simulink model "gnc_PathTracker"  (R2026b)
settings: Solver=VariableStepAuto
values from neighbouring files (symbols this model uses):
  Ts = prm.Ts    [gnc_missionFSM.m]    (also in gnc_mpcPlantUpdate.m)
undefined symbols (not defined in the file or in its folder): P
libraries: robotalgslib x1, mpclib x1, drivingvehiclecontroller x1, simulink x1
settings Model: Creator=aomar  LastModifiedBy=aomar

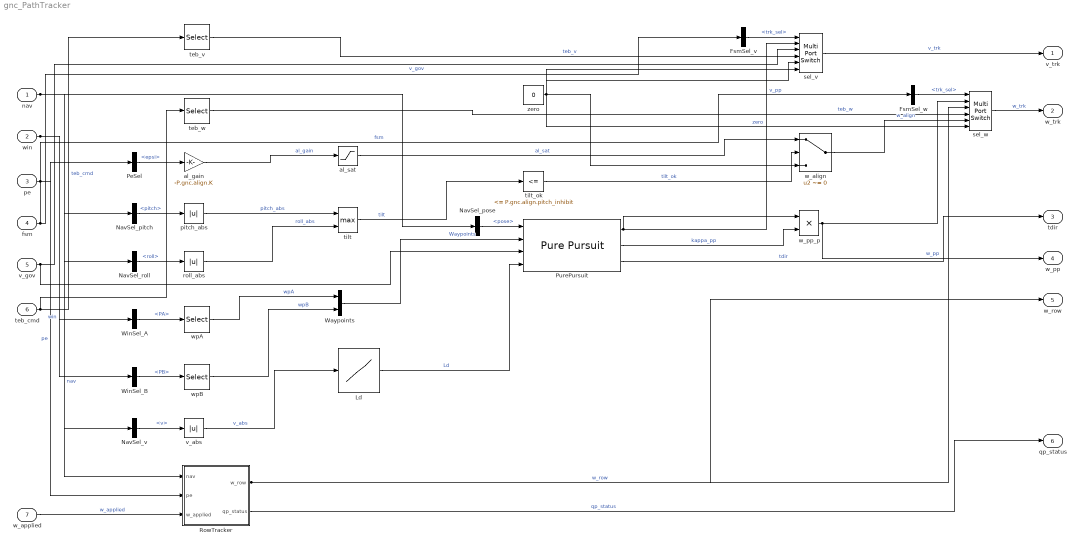
== system gnc_PathTracker ==
  nav : Inport  OutDataTypeStr=Bus: Bus_NavCond  SampleTime=Ts.gnc
  win : Inport  Port=2  OutDataTypeStr=Bus: Bus_PathWindow  SampleTime=Ts.gnc
  pe : Inport  Port=3  OutDataTypeStr=Bus: Bus_PathError  SampleTime=Ts.gnc
  fsm : Inport  Port=4  OutDataTypeStr=Bus: Bus_FsmOut  SampleTime=Ts.gnc
  v_gov : Inport  Port=5  OutDataTypeStr=double  PortDimensions=1  SampleTime=Ts.gnc
  teb_cmd : Inport  Port=6  OutDataTypeStr=double  PortDimensions=2  SampleTime=Ts.gnc
  w_applied : Inport  Port=7  OutDataTypeStr=double  PortDimensions=1  SampleTime=Ts.gnc
  FsmSel_v : BusSelector  OutputSignals=trk_sel
  FsmSel_w : BusSelector  OutputSignals=trk_sel
  Ld : Lookup_n-D  NumberOfTableDimensions=1  BreakpointsForDimension1=P.gnc.pp.Ld_v  Table=P.gnc.pp.Ld  ExtrapMethod=Clip  UseLastTableValue=on  InternalRulePriority=Speed  RndMeth=Simplest
  NavSel_pitch : BusSelector  OutputSignals=pitch
  NavSel_pose : BusSelector  OutputSignals=pose
  NavSel_roll : BusSelector  OutputSignals=roll
  NavSel_v : BusSelector  OutputSignals=v
  PeSel : BusSelector  OutputSignals=epsi
  PurePursuit : robotalgslib/Pure Pursuit  DesiredLinearVelocityPort=on  DesiredLinearVelocity=0.1  MaxCurvature=P.gnc.pp.kappa_max  LookaheadDistancePort=on  LookaheadDistance=1.0  TargetDirPort=on  SimulateUsing=Code generation
      settings: LibrarySourceBlock=robotmobilelib/Pure Pursuit
  RowTracker : Subsystem  Variant=on
  Waypoints : Concatenate  Mode=Multidimensional array
  WinSel_A : BusSelector  OutputSignals=PA
  WinSel_B : BusSelector  OutputSignals=PB
  al_gain : Gain  Gain=-P.gnc.align.K
  al_sat : Saturate  UpperLimit=P.gnc.align.w_max  LowerLimit=-P.gnc.align.w_max
  pitch_abs : Abs  SaturateOnIntegerOverflow=off
  roll_abs : Abs  SaturateOnIntegerOverflow=off
  sel_v : MultiPortSwitch  DataPortOrder=Specify indices  Inputs=5  DataPortIndices={1,2,3,4,0}  DiagnosticForDefault=None  SaturateOnIntegerOverflow=off  InputSameDT=off
  sel_w : MultiPortSwitch  DataPortOrder=Specify indices  Inputs=5  DataPortIndices={1,2,3,4,0}  DiagnosticForDefault=None  SaturateOnIntegerOverflow=off  InputSameDT=off
  teb_v : Selector  IndexOptions=Index vector (dialog)  Indices=1  OutputSizes=1
  teb_w : Selector  IndexOptions=Index vector (dialog)  Indices=2  OutputSizes=1
  tilt : MinMax  Function=max  Inputs=2
  tilt_ok : simulink/Logic and Bit Operations/Compare To Constant  relop=<=  const=P.gnc.align.pitch_inhibit  OutDataTypeStr=boolean
  v_abs : Abs  SaturateOnIntegerOverflow=off
  w_align : Switch  Criteria=u2 ~= 0  SaturateOnIntegerOverflow=off  InputSameDT=off
  w_pp_p : Product  Inputs=**
  wpA : Selector  NumberOfDimensions=2  InputPortWidth=3  IndexOptions=Select all,Index vector (dialog)  Indices=,[1 2]  OutputSizes=1
  wpB : Selector  NumberOfDimensions=2  InputPortWidth=3  IndexOptions=Index vector (dialog),Index vector (dialog)  Indices=2:P.gnc.path.N_smooth,[1 2]  OutputSizes=1
  zero : Constant  Value=0  OutDataTypeStr=double  SampleTime=Ts.gnc
  v_trk : Outport  OutDataTypeStr=double
  w_trk : Outport  Port=2  OutDataTypeStr=double
  tdir : Outport  Port=3  OutDataTypeStr=double
  w_pp : Outport  Port=4  OutDataTypeStr=double
  w_row : Outport  Port=5  OutDataTypeStr=double
  qp_status : Outport  Port=6  OutDataTypeStr=int32
  wires:
  win/1 -> WinSel_B/1, WinSel_A/1  "win"
  v_gov/1 -> sel_v/3, PurePursuit/3  "v_gov"
  teb_cmd/1 -> teb_v/1, teb_w/1  "teb_cmd"
  w_applied/1 -> RowTracker/3(w_applied)  "w_applied"
  PeSel/1 -> al_gain/1  "<epsi>"
  NavSel_pitch/1 -> pitch_abs/1  "<pitch>"
  NavSel_roll/1 -> roll_abs/1  "<roll>"
  WinSel_A/1 -> wpA/1  "<PA>"
  WinSel_B/1 -> wpB/1  "<PB>"
  NavSel_v/1 -> v_abs/1  "<v>"
  al_gain/1 -> al_sat/1  "al_gain"
  pitch_abs/1 -> tilt/1  "pitch_abs"
  roll_abs/1 -> tilt/2  "roll_abs"
  v_abs/1 -> Ld/1  "v_abs"
  teb_v/1 -> sel_v/4  "teb_v"
  teb_w/1 -> sel_w/4  "teb_w"
  wpA/1 -> Waypoints/1  "wpA"
  wpB/1 -> Waypoints/2  "wpB"
  RowTracker/1(w_row) -> sel_w/3, w_row/1  "w_row"
  RowTracker/2(qp_status) -> qp_status/1  "qp_status"
  Waypoints/1 -> PurePursuit/2  "Waypoints"
  al_sat/1 -> w_align/1  "al_sat"
  tilt/1 -> tilt_ok/1  "tilt"
  Ld/1 -> PurePursuit/4  "Ld"
  NavSel_pose/1 -> PurePursuit/1  "<pose>"
  zero/1 -> w_align/3, sel_v/5, sel_w/6, sel_v/6  "zero"
  tilt_ok/1 -> w_align/2  "tilt_ok"
  PurePursuit/1 -> sel_v/2, w_pp_p/1  "v_pp"
  PurePursuit/2 -> w_pp_p/2  "kappa_pp"
  PurePursuit/3 -> tdir/1  "tdir"
  FsmSel_v/1 -> sel_v/1  "<trk_sel>"
  w_pp_p/1 -> sel_w/2, w_pp/1  "w_pp"
  sel_v/1 -> v_trk/1  "v_trk"
  w_align/1 -> sel_w/5  "w_align"
  FsmSel_w/1 -> sel_w/1  "<trk_sel>"
  sel_w/1 -> w_trk/1  "w_trk"
  pe/1 -> PeSel/1, RowTracker/2(pe)  "pe"
  fsm/1 -> FsmSel_v/1, FsmSel_w/1  "fsm"
  nav/1 -> RowTracker/1(nav), NavSel_v/1, NavSel_roll/1, NavSel_pose/1, NavSel_pitch/1  "nav"

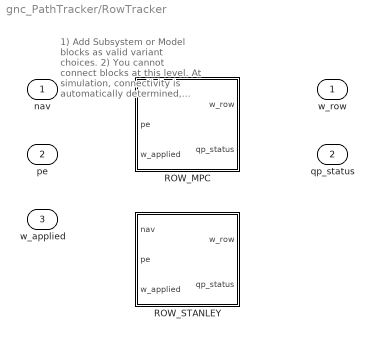
== system gnc_PathTracker/RowTracker ==
  note: 1) Add Subsystem or Model blocks as valid variant choices.
      | 2) You cannot connect blocks at this level. At simulation, connectivity is automatically
      | determined, based on the active variant and port name matching.
  nav : Inport
  pe : Inport  Port=2
  w_applied : Inport  Port=3
  ROW_MPC : Subsystem  VariantControl=VC_ROW_TRACKER == 1
  ROW_STANLEY : Subsystem  VariantControl=VC_ROW_TRACKER == 2
  w_row : Outport
  qp_status : Outport  Port=2

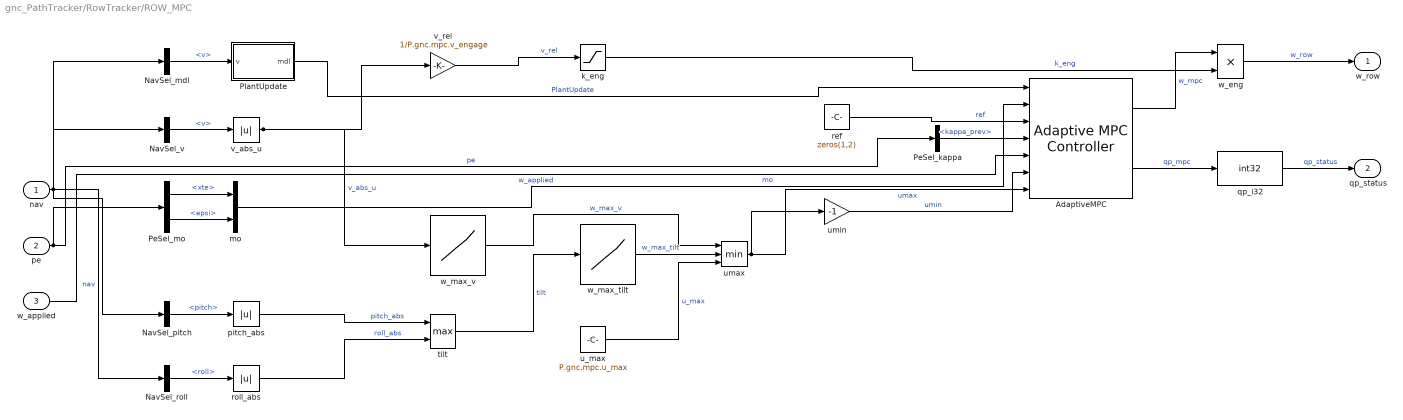
== system gnc_PathTracker/RowTracker/ROW_MPC ==
  nav : Inport
  pe : Inport  Port=2
  w_applied : Inport  Port=3
  AdaptiveMPC : mpclib/Adaptive MPC Controller  SCDEnableBlockLinearizationSpecification=on  mpcobj=mpcRowObj  enable_value=0  updateMPCinCallerWorkspace=on  md_inport=on  mv_inport=on  uref_inport=off  return_cost=off  return_mvseq=off  return_qpstatus=on  return_xseq=off  return_state=off  return_ovseq=off  state_inport=off  isltv_plant=off  umin_inport=on  umax_inport=on  ymin_inport=off  ymax_inport=off  cc_inport=off  ywt_inport=off  uwt_inport=off  duwt_inport=off  rhoeps_inport=off  pm_inport=off  MaximumP=10  HorizonChoice=FixedHorizon  BlockDataType=double  SampleTimeInherited=off  switch_inport=off
  NavSel_mdl : BusSelector  OutputSignals=v
  NavSel_pitch : BusSelector  OutputSignals=pitch
  NavSel_roll : BusSelector  OutputSignals=roll
  NavSel_v : BusSelector  OutputSignals=v
  PeSel_kappa : BusSelector  OutputSignals=kappa_prev
  PeSel_mo : BusSelector  OutputSignals=xte,epsi
  PlantUpdate : MATLAB Function  TreatAsAtomicUnit=on  mask{mpc=P.gnc.mpc}
  k_eng : Saturate  UpperLimit=1  LowerLimit=0
  mo : Mux  Inputs=2
  pitch_abs : Abs  SaturateOnIntegerOverflow=off
  qp_i32 : DataTypeConversion  OutDataTypeStr=int32  RndMeth=Nearest
  ref : Constant  Value=zeros(1,2)  OutDataTypeStr=double  SampleTime=Ts.gnc
  roll_abs : Abs  SaturateOnIntegerOverflow=off
  tilt : MinMax  Function=max  Inputs=2
  u_max : Constant  Value=P.gnc.mpc.u_max  OutDataTypeStr=double  SampleTime=Ts.gnc
  umax : MinMax  Inputs=3
  umin : Gain  Gain=-1
  v_abs_u : Abs  SaturateOnIntegerOverflow=off
  v_rel : Gain  Gain=1/P.gnc.mpc.v_engage
  w_eng : Product  Inputs=**
  w_max_tilt : Lookup_n-D  NumberOfTableDimensions=1  BreakpointsForDimension1=P.gnc.cmd.w_tilt_x  Table=P.gnc.cmd.w_tilt  ExtrapMethod=Clip  UseLastTableValue=on  InternalRulePriority=Speed  RndMeth=Simplest
  w_max_v : Lookup_n-D  NumberOfTableDimensions=1  BreakpointsForDimension1=P.gnc.cmd.w_max_v  Table=P.gnc.cmd.w_max  ExtrapMethod=Clip  UseLastTableValue=on  InternalRulePriority=Speed  RndMeth=Simplest
  w_row : Outport
  qp_status : Outport  Port=2
  wires:
  nav/1 -> NavSel_roll/1, NavSel_mdl/1, NavSel_pitch/1, NavSel_v/1  "nav"
  pe/1 -> PeSel_kappa/1, PeSel_mo/1  "pe"
  w_applied/1 -> AdaptiveMPC/5  "w_applied"
  NavSel_mdl/1 -> PlantUpdate/1(v)  "<v>"
  NavSel_v/1 -> v_abs_u/1  "<v>"
  PeSel_mo/1 -> mo/1  "<xte>"
  PeSel_mo/2 -> mo/2  "<epsi>"
  NavSel_pitch/1 -> pitch_abs/1  "<pitch>"
  NavSel_roll/1 -> roll_abs/1  "<roll>"
  mo/1 -> AdaptiveMPC/2  "mo"
  v_abs_u/1 -> w_max_v/1, v_rel/1  "v_abs_u"
  pitch_abs/1 -> tilt/1  "pitch_abs"
  roll_abs/1 -> tilt/2  "roll_abs"
  PlantUpdate/1(mdl) -> AdaptiveMPC/1  "PlantUpdate"
  v_rel/1 -> k_eng/1  "v_rel"
  tilt/1 -> w_max_tilt/1  "tilt"
  w_max_v/1 -> umax/1  "w_max_v"
  k_eng/1 -> w_eng/2  "k_eng"
  u_max/1 -> umax/3  "u_max"
  w_max_tilt/1 -> umax/2  "w_max_tilt"
  umax/1 -> AdaptiveMPC/7, umin/1  "umax"
  ref/1 -> AdaptiveMPC/3  "ref"
  umin/1 -> AdaptiveMPC/6  "umin"
  PeSel_kappa/1 -> AdaptiveMPC/4  "<kappa_prev>"
  AdaptiveMPC/1 -> w_eng/1  "w_mpc"
  AdaptiveMPC/2 -> qp_i32/1  "qp_mpc"
  w_eng/1 -> w_row/1  "w_row"
  qp_i32/1 -> qp_status/1  "qp_status"

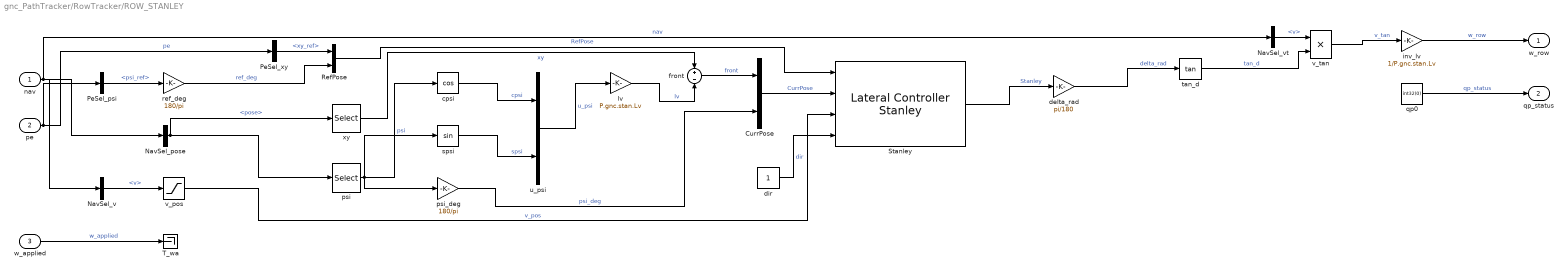
== system gnc_PathTracker/RowTracker/ROW_STANLEY ==
  nav : Inport
  pe : Inport  Port=2
  w_applied : Inport  Port=3
  CurrPose : Concatenate
  NavSel_pose : BusSelector  OutputSignals=pose
  NavSel_v : BusSelector  OutputSignals=v
  NavSel_vt : BusSelector  OutputSignals=v
  PeSel_psi : BusSelector  OutputSignals=psi_ref
  PeSel_xy : BusSelector  OutputSignals=xy_ref
  RefPose : Concatenate
  Stanley : drivingvehiclecontroller/Lateral Controller Stanley  ModelType=Kinematic bicycle model  PositionGainF=P.gnc.stan.k_block  PositionGainR=P.gnc.stan.k_block  YawRateGain=0.2  DelayGain=0.2  VehicleMass=1575  Lf=1.2  Lr=1.6  TireStiffness=19000  Wheelbase=P.gnc.stan.Lv  MaxSteeringAngle=P.gnc.stan.delta_max_deg
  T_wa : Terminator
  cpsi : Trigonometry  Operator=cos
  delta_rad : Gain  Gain=pi/180
  dir : Constant  OutDataTypeStr=double  SampleTime=Ts.gnc
  front : Sum  Inputs=+-
  inv_lv : Gain  Gain=1/P.gnc.stan.Lv
  lv : Gain  Gain=P.gnc.stan.Lv
  psi : Selector  IndexOptions=Index vector (dialog)  Indices=3  OutputSizes=1
  psi_deg : Gain  Gain=180/pi
  qp0 : Constant  Value=int32(0)  OutDataTypeStr=int32  SampleTime=Ts.gnc
  ref_deg : Gain  Gain=180/pi
  spsi : Trigonometry
  tan_d : Trigonometry  Operator=tan
  u_psi : Mux  Inputs=2
  v_pos : Saturate  UpperLimit=inf  LowerLimit=P.gnc.mpc.v_min_model
  v_tan : Product  Inputs=**
  xy : Selector  IndexOptions=Index vector (dialog)  Indices=[1 2]  OutputSizes=1
  w_row : Outport
  qp_status : Outport  Port=2
  wires:
  w_applied/1 -> T_wa/1  "w_applied"
  PeSel_psi/1 -> ref_deg/1  "<psi_ref>"
  NavSel_v/1 -> v_pos/1  "<v>"
  NavSel_pose/1 -> psi/1, xy/1  "<pose>"
  ref_deg/1 -> RefPose/2  "ref_deg"
  v_pos/1 -> Stanley/3  "v_pos"
  PeSel_xy/1 -> RefPose/1  "<xy_ref>"
  RefPose/1 -> Stanley/1  "RefPose"
  xy/1 -> front/1  "xy"
  psi/1 -> cpsi/1, spsi/1, psi_deg/1  "psi"
  cpsi/1 -> u_psi/1  "cpsi"
  spsi/1 -> u_psi/2  "spsi"
  psi_deg/1 -> CurrPose/2  "psi_deg"
  u_psi/1 -> lv/1  "u_psi"
  lv/1 -> front/2  "lv"
  front/1 -> CurrPose/1  "front"
  CurrPose/1 -> Stanley/2  "CurrPose"
  dir/1 -> Stanley/4  "dir"
  Stanley/1 -> delta_rad/1  "Stanley"
  delta_rad/1 -> tan_d/1  "delta_rad"
  tan_d/1 -> v_tan/2  "tan_d"
  NavSel_vt/1 -> v_tan/1  "<v>"
  v_tan/1 -> inv_lv/1  "v_tan"
  inv_lv/1 -> w_row/1  "w_row"
  qp0/1 -> qp_status/1  "qp_status"
  nav/1 -> NavSel_v/1, NavSel_pose/1, NavSel_vt/1  "nav"
  pe/1 -> PeSel_xy/1, PeSel_psi/1  "pe"

== matlab function gnc_PathTracker/RowTracker/ROW_MPC/PlantUpdate ==
  settings: updateMethod=DISCRETE  sampleTime=Ts.gnc  description=LTV prediction model for the Adaptive MPC model inport (gnc spec 4.3, D41); body subsystems/gnc/gnc_mpcPlantUpdate.m.
  data: v input; mdl output Bus: Bus_MpcModel; mpc parameter
function mdl = fcn(v, mpc)
%#codegen
mdl = gnc_mpcPlantUpdate(v, mpc);
